simulink model "tb_drive_sys"  (R2026b)
settings: Solver=ode3  StopTime=1  FixedStep=1e-3  EnableMultiTasking=on
model workspace (MAT data in the model file):
  tb_J = 1.2798
  tb_Rsrc = 0.02
  tb_T_amb = 318.15
  tb_Trr = 6.97491
  tb_cmd.enable = timeseries
  tb_cmd.enable.Name = 'unnamed'
  tb_cmd.enable.DataInfo = tsdata.datametadata
  tb_cmd.enable.DataInfo.Interpolation = tsdata.interpolation
  tb_cmd.enable.DataInfo.Interpolation.Fhandle : function handle (value not decoded)
  tb_cmd.enable.DataInfo.Interpolation.Name = 'linear'
  tb_cmd.enable.TimeInfo = tsdata.timemetadata
  tb_cmd.enable.TimeInfo.Length = 1
  tb_cmd.enable.TimeInfo.DuplicateTimes = 0
  tb_cmd.enable.TimeInfo.Time_ = 0
  tb_cmd.enable.TimeInfo.Initialized = 1
  tb_cmd.enable.QualityInfo = tsdata.qualmetadata
  tb_cmd.enable.Data_ = 0
  tb_cmd.mode = timeseries
  tb_cmd.mode.Name = 'unnamed'
  tb_cmd.mode.DataInfo = tsdata.datametadata
  tb_cmd.mode.DataInfo.Interpolation = tsdata.interpolation
  tb_cmd.mode.DataInfo.Interpolation.Fhandle : function handle (value not decoded)
  tb_cmd.mode.DataInfo.Interpolation.Name = 'linear'
  tb_cmd.mode.TimeInfo = tsdata.timemetadata
  tb_cmd.mode.TimeInfo.Length = 1
  tb_cmd.mode.TimeInfo.DuplicateTimes = 0
  tb_cmd.mode.TimeInfo.Time_ = 0
  tb_cmd.mode.TimeInfo.Initialized = 1
  tb_cmd.mode.QualityInfo = tsdata.qualmetadata
  tb_cmd.mode.Data_ = 1
  tb_cmd.w_ref = timeseries
  tb_cmd.w_ref.Name = 'unnamed'
  tb_cmd.w_ref.DataInfo = tsdata.datametadata
  tb_cmd.w_ref.DataInfo.Interpolation = tsdata.interpolation
  tb_cmd.w_ref.DataInfo.Interpolation.Fhandle : function handle (value not decoded)
  tb_cmd.w_ref.DataInfo.Interpolation.Name = 'linear'
  tb_cmd.w_ref.TimeInfo = tsdata.timemetadata
  tb_cmd.w_ref.TimeInfo.Length = 1
  tb_cmd.w_ref.TimeInfo.DuplicateTimes = 0
  tb_cmd.w_ref.TimeInfo.Time_ = 0
  tb_cmd.w_ref.TimeInfo.Initialized = 1
  tb_cmd.w_ref.QualityInfo = tsdata.qualmetadata
  tb_cmd.w_ref.Data_ = 0
  tb_cmd.tau_ff = timeseries
  tb_cmd.tau_ff.Name = 'unnamed'
  tb_cmd.tau_ff.DataInfo = tsdata.datametadata
  tb_cmd.tau_ff.DataInfo.Interpolation = tsdata.interpolation
  tb_cmd.tau_ff.DataInfo.Interpolation.Fhandle : function handle (value not decoded)
  tb_cmd.tau_ff.DataInfo.Interpolation.Name = 'linear'
  tb_cmd.tau_ff.TimeInfo = tsdata.timemetadata
  tb_cmd.tau_ff.TimeInfo.Length = 1
  tb_cmd.tau_ff.TimeInfo.DuplicateTimes = 0
  tb_cmd.tau_ff.TimeInfo.Time_ = 0
  tb_cmd.tau_ff.TimeInfo.Initialized = 1
  tb_cmd.tau_ff.QualityInfo = tsdata.qualmetadata
  tb_cmd.tau_ff.Data_ = 0
  tb_cmd.tau_lim_mot = timeseries
  tb_cmd.tau_lim_mot.Name = 'unnamed'
  tb_cmd.tau_lim_mot.DataInfo = tsdata.datametadata
  tb_cmd.tau_lim_mot.DataInfo.Interpolation = tsdata.interpolation
  tb_cmd.tau_lim_mot.DataInfo.Interpolation.Fhandle : function handle (value not decoded)
  tb_cmd.tau_lim_mot.DataInfo.Interpolation.Name = 'linear'
  tb_cmd.tau_lim_mot.TimeInfo = tsdata.timemetadata
  tb_cmd.tau_lim_mot.TimeInfo.Length = 1
  tb_cmd.tau_lim_mot.TimeInfo.DuplicateTimes = 0
  tb_cmd.tau_lim_mot.TimeInfo.Time_ = 0
  tb_cmd.tau_lim_mot.TimeInfo.Initialized = 1
  tb_cmd.tau_lim_mot.QualityInfo = tsdata.qualmetadata
  tb_cmd.tau_lim_mot.Data_ = 16
  tb_cmd.tau_lim_reg = timeseries
  tb_cmd.tau_lim_reg.Name = 'unnamed'
  tb_cmd.tau_lim_reg.DataInfo = tsdata.datametadata
  tb_cmd.tau_lim_reg.DataInfo.Interpolation = tsdata.interpolation
  tb_cmd.tau_lim_reg.DataInfo.Interpolation.Fhandle : function handle (value not decoded)
  tb_cmd.tau_lim_reg.DataInfo.Interpolation.Name = 'linear'
  tb_cmd.tau_lim_reg.TimeInfo = tsdata.timemetadata
  tb_cmd.tau_lim_reg.TimeInfo.Length = 1
  tb_cmd.tau_lim_reg.TimeInfo.DuplicateTimes = 0
  tb_cmd.tau_lim_reg.TimeInfo.Time_ = 0
  tb_cmd.tau_lim_reg.TimeInfo.Initialized = 1
  tb_cmd.tau_lim_reg.QualityInfo = tsdata.qualmetadata
  tb_cmd.tau_lim_reg.Data_ = 16
  tb_cmd.park_req = timeseries
  tb_cmd.park_req.Name = 'unnamed'
  tb_cmd.park_req.DataInfo = tsdata.datametadata
  tb_cmd.park_req.DataInfo.Interpolation = tsdata.interpolation
  tb_cmd.park_req.DataInfo.Interpolation.Fhandle : function handle (value not decoded)
  tb_cmd.park_req.DataInfo.Interpolation.Name = 'linear'
  tb_cmd.park_req.TimeInfo = tsdata.timemetadata
  tb_cmd.park_req.TimeInfo.Length = 1
  tb_cmd.park_req.TimeInfo.DuplicateTimes = 0
  tb_cmd.park_req.TimeInfo.Time_ = 0
  tb_cmd.park_req.TimeInfo.Initialized = 1
  tb_cmd.park_req.QualityInfo = tsdata.qualmetadata
  tb_cmd.park_req.Data_ = 0
  tb_cmd.fault_reset = timeseries
  tb_cmd.fault_reset.Name = 'unnamed'
  tb_cmd.fault_reset.DataInfo = tsdata.datametadata
  tb_cmd.fault_reset.DataInfo.Interpolation = tsdata.interpolation
  tb_cmd.fault_reset.DataInfo.Interpolation.Fhandle : function handle (value not decoded)
  tb_cmd.fault_reset.DataInfo.Interpolation.Name = 'linear'
  tb_cmd.fault_reset.TimeInfo = tsdata.timemetadata
  tb_cmd.fault_reset.TimeInfo.Length = 1
  tb_cmd.fault_reset.TimeInfo.DuplicateTimes = 0
  tb_cmd.fault_reset.TimeInfo.Time_ = 0
  tb_cmd.fault_reset.TimeInfo.Initialized = 1
  tb_cmd.fault_reset.QualityInfo = tsdata.qualmetadata
  tb_cmd.fault_reset.Data_ = 0
  tb_cmd.alive = timeseries
  tb_cmd.alive.Name = 'unnamed'
  tb_cmd.alive.DataInfo = tsdata.datametadata
  tb_cmd.alive.DataInfo.Interpolation = tsdata.interpolation
  tb_cmd.alive.DataInfo.Interpolation.Fhandle : function handle (value not decoded)
  tb_cmd.alive.DataInfo.Interpolation.Name = 'linear'
  tb_cmd.alive.TimeInfo = tsdata.timemetadata
  tb_cmd.alive.TimeInfo.Length = 1
  tb_cmd.alive.TimeInfo.DuplicateTimes = 0
  tb_cmd.alive.TimeInfo.Time_ = 0
  tb_cmd.alive.TimeInfo.Initialized = 1
  tb_cmd.alive.QualityInfo = tsdata.qualmetadata
  tb_cmd.alive.Data_ = 0
  tb_cmdL.enable = timeseries
  tb_cmdL.enable.Name = 'unnamed'
  tb_cmdL.enable.DataInfo = tsdata.datametadata
  tb_cmdL.enable.DataInfo.Interpolation = tsdata.interpolation
  tb_cmdL.enable.DataInfo.Interpolation.Fhandle : function handle (value not decoded)
  tb_cmdL.enable.DataInfo.Interpolation.Name = 'linear'
  tb_cmdL.enable.TimeInfo = tsdata.timemetadata
  tb_cmdL.enable.TimeInfo.Length = 1
  tb_cmdL.enable.TimeInfo.DuplicateTimes = 0
  tb_cmdL.enable.TimeInfo.Time_ = 0
  tb_cmdL.enable.TimeInfo.Initialized = 1
  tb_cmdL.enable.QualityInfo = tsdata.qualmetadata
  tb_cmdL.enable.Data_ = 0
  tb_cmdL.mode = timeseries
  tb_cmdL.mode.Name = 'unnamed'
  tb_cmdL.mode.DataInfo = tsdata.datametadata
  tb_cmdL.mode.DataInfo.Interpolation = tsdata.interpolation
  tb_cmdL.mode.DataInfo.Interpolation.Fhandle : function handle (value not decoded)
  tb_cmdL.mode.DataInfo.Interpolation.Name = 'linear'
  tb_cmdL.mode.TimeInfo = tsdata.timemetadata
  tb_cmdL.mode.TimeInfo.Length = 1
  tb_cmdL.mode.TimeInfo.DuplicateTimes = 0
  tb_cmdL.mode.TimeInfo.Time_ = 0
  tb_cmdL.mode.TimeInfo.Initialized = 1
  tb_cmdL.mode.QualityInfo = tsdata.qualmetadata
  tb_cmdL.mode.Data_ = 1
  tb_cmdL.w_ref = timeseries
  tb_cmdL.w_ref.Name = 'unnamed'
  tb_cmdL.w_ref.DataInfo = tsdata.datametadata
  tb_cmdL.w_ref.DataInfo.Interpolation = tsdata.interpolation
  tb_cmdL.w_ref.DataInfo.Interpolation.Fhandle : function handle (value not decoded)
  tb_cmdL.w_ref.DataInfo.Interpolation.Name = 'linear'
  tb_cmdL.w_ref.TimeInfo = tsdata.timemetadata
  tb_cmdL.w_ref.TimeInfo.Length = 1
  tb_cmdL.w_ref.TimeInfo.DuplicateTimes = 0
  tb_cmdL.w_ref.TimeInfo.Time_ = 0
  tb_cmdL.w_ref.TimeInfo.Initialized = 1
  tb_cmdL.w_ref.QualityInfo = tsdata.qualmetadata
  tb_cmdL.w_ref.Data_ = 0
  tb_cmdL.tau_ff = timeseries
  tb_cmdL.tau_ff.Name = 'unnamed'
  tb_cmdL.tau_ff.DataInfo = tsdata.datametadata
  tb_cmdL.tau_ff.DataInfo.Interpolation = tsdata.interpolation
  tb_cmdL.tau_ff.DataInfo.Interpolation.Fhandle : function handle (value not decoded)
  tb_cmdL.tau_ff.DataInfo.Interpolation.Name = 'linear'
  tb_cmdL.tau_ff.TimeInfo = tsdata.timemetadata
  tb_cmdL.tau_ff.TimeInfo.Length = 1
  tb_cmdL.tau_ff.TimeInfo.DuplicateTimes = 0
  tb_cmdL.tau_ff.TimeInfo.Time_ = 0
  tb_cmdL.tau_ff.TimeInfo.Initialized = 1
  tb_cmdL.tau_ff.QualityInfo = tsdata.qualmetadata
  tb_cmdL.tau_ff.Data_ = 0
  tb_cmdL.tau_lim_mot = timeseries
  tb_cmdL.tau_lim_mot.Name = 'unnamed'
  tb_cmdL.tau_lim_mot.DataInfo = tsdata.datametadata
  tb_cmdL.tau_lim_mot.DataInfo.Interpolation = tsdata.interpolation
  tb_cmdL.tau_lim_mot.DataInfo.Interpolation.Fhandle : function handle (value not decoded)
  tb_cmdL.tau_lim_mot.DataInfo.Interpolation.Name = 'linear'
  tb_cmdL.tau_lim_mot.TimeInfo = tsdata.timemetadata
  tb_cmdL.tau_lim_mot.TimeInfo.Length = 1
  tb_cmdL.tau_lim_mot.TimeInfo.DuplicateTimes = 0
  tb_cmdL.tau_lim_mot.TimeInfo.Time_ = 0
  tb_cmdL.tau_lim_mot.TimeInfo.Initialized = 1
  tb_cmdL.tau_lim_mot.QualityInfo = tsdata.qualmetadata
  tb_cmdL.tau_lim_mot.Data_ = 16
  tb_cmdL.tau_lim_reg = timeseries
  tb_cmdL.tau_lim_reg.Name = 'unnamed'
  tb_cmdL.tau_lim_reg.DataInfo = tsdata.datametadata
  tb_cmdL.tau_lim_reg.DataInfo.Interpolation = tsdata.interpolation
  tb_cmdL.tau_lim_reg.DataInfo.Interpolation.Fhandle : function handle (value not decoded)
  tb_cmdL.tau_lim_reg.DataInfo.Interpolation.Name = 'linear'
  tb_cmdL.tau_lim_reg.TimeInfo = tsdata.timemetadata
  tb_cmdL.tau_lim_reg.TimeInfo.Length = 1
  tb_cmdL.tau_lim_reg.TimeInfo.DuplicateTimes = 0
  tb_cmdL.tau_lim_reg.TimeInfo.Time_ = 0
  tb_cmdL.tau_lim_reg.TimeInfo.Initialized = 1
  tb_cmdL.tau_lim_reg.QualityInfo = tsdata.qualmetadata
  tb_cmdL.tau_lim_reg.Data_ = 16
  tb_cmdL.park_req = timeseries
  tb_cmdL.park_req.Name = 'unnamed'
  tb_cmdL.park_req.DataInfo = tsdata.datametadata
  tb_cmdL.park_req.DataInfo.Interpolation = tsdata.interpolation
  tb_cmdL.park_req.DataInfo.Interpolation.Fhandle : function handle (value not decoded)
  tb_cmdL.park_req.DataInfo.Interpolation.Name = 'linear'
  tb_cmdL.park_req.TimeInfo = tsdata.timemetadata
  tb_cmdL.park_req.TimeInfo.Length = 1
  tb_cmdL.park_req.TimeInfo.DuplicateTimes = 0
  tb_cmdL.park_req.TimeInfo.Time_ = 0
  tb_cmdL.park_req.TimeInfo.Initialized = 1
  tb_cmdL.park_req.QualityInfo = tsdata.qualmetadata
  tb_cmdL.park_req.Data_ = 0
  tb_cmdL.fault_reset = timeseries
  tb_cmdL.fault_reset.Name = 'unnamed'
  tb_cmdL.fault_reset.DataInfo = tsdata.datametadata
  tb_cmdL.fault_reset.DataInfo.Interpolation = tsdata.interpolation
  tb_cmdL.fault_reset.DataInfo.Interpolation.Fhandle : function handle (value not decoded)
  tb_cmdL.fault_reset.DataInfo.Interpolation.Name = 'linear'
  tb_cmdL.fault_reset.TimeInfo = tsdata.timemetadata
  tb_cmdL.fault_reset.TimeInfo.Length = 1
  tb_cmdL.fault_reset.TimeInfo.DuplicateTimes = 0
  tb_cmdL.fault_reset.TimeInfo.Time_ = 0
  tb_cmdL.fault_reset.TimeInfo.Initialized = 1
  tb_cmdL.fault_reset.QualityInfo = tsdata.qualmetadata
  tb_cmdL.fault_reset.Data_ = 0
  tb_cmdL.alive = timeseries
  tb_cmdL.alive.Name = 'unnamed'
  tb_cmdL.alive.DataInfo = tsdata.datametadata
  tb_cmdL.alive.DataInfo.Interpolation = tsdata.interpolation
  tb_cmdL.alive.DataInfo.Interpolation.Fhandle : function handle (value not decoded)
  tb_cmdL.alive.DataInfo.Interpolation.Name = 'linear'
  tb_cmdL.alive.TimeInfo = tsdata.timemetadata
  tb_cmdL.alive.TimeInfo.Length = 1
  tb_cmdL.alive.TimeInfo.DuplicateTimes = 0
  tb_cmdL.alive.TimeInfo.Time_ = 0
  tb_cmdL.alive.TimeInfo.Initialized = 1
  tb_cmdL.alive.QualityInfo = tsdata.qualmetadata
  tb_cmdL.alive.Data_ = 0
  tb_cmdR.enable = timeseries
  tb_cmdR.enable.Name = 'unnamed'
  tb_cmdR.enable.DataInfo = tsdata.datametadata
  tb_cmdR.enable.DataInfo.Interpolation = tsdata.interpolation
  tb_cmdR.enable.DataInfo.Interpolation.Fhandle : function handle (value not decoded)
  tb_cmdR.enable.DataInfo.Interpolation.Name = 'linear'
  tb_cmdR.enable.TimeInfo = tsdata.timemetadata
  tb_cmdR.enable.TimeInfo.Length = 1
  tb_cmdR.enable.TimeInfo.DuplicateTimes = 0
  tb_cmdR.enable.TimeInfo.Time_ = 0
  tb_cmdR.enable.TimeInfo.Initialized = 1
  tb_cmdR.enable.QualityInfo = tsdata.qualmetadata
  tb_cmdR.enable.Data_ = 0
  tb_cmdR.mode = timeseries
  tb_cmdR.mode.Name = 'unnamed'
  tb_cmdR.mode.DataInfo = tsdata.datametadata
  tb_cmdR.mode.DataInfo.Interpolation = tsdata.interpolation
  tb_cmdR.mode.DataInfo.Interpolation.Fhandle : function handle (value not decoded)
  tb_cmdR.mode.DataInfo.Interpolation.Name = 'linear'
  tb_cmdR.mode.TimeInfo = tsdata.timemetadata
  tb_cmdR.mode.TimeInfo.Length = 1
  tb_cmdR.mode.TimeInfo.DuplicateTimes = 0
  tb_cmdR.mode.TimeInfo.Time_ = 0
  tb_cmdR.mode.TimeInfo.Initialized = 1
  tb_cmdR.mode.QualityInfo = tsdata.qualmetadata
  tb_cmdR.mode.Data_ = 1
  tb_cmdR.w_ref = timeseries
  tb_cmdR.w_ref.Name = 'unnamed'
  tb_cmdR.w_ref.DataInfo = tsdata.datametadata
  tb_cmdR.w_ref.DataInfo.Interpolation = tsdata.interpolation
  tb_cmdR.w_ref.DataInfo.Interpolation.Fhandle : function handle (value not decoded)
  tb_cmdR.w_ref.DataInfo.Interpolation.Name = 'linear'
  tb_cmdR.w_ref.TimeInfo = tsdata.timemetadata
  tb_cmdR.w_ref.TimeInfo.Length = 1
  tb_cmdR.w_ref.TimeInfo.DuplicateTimes = 0
  tb_cmdR.w_ref.TimeInfo.Time_ = 0
  tb_cmdR.w_ref.TimeInfo.Initialized = 1
  tb_cmdR.w_ref.QualityInfo = tsdata.qualmetadata
  tb_cmdR.w_ref.Data_ = 0
  tb_cmdR.tau_ff = timeseries
  tb_cmdR.tau_ff.Name = 'unnamed'
  tb_cmdR.tau_ff.DataInfo = tsdata.datametadata
  tb_cmdR.tau_ff.DataInfo.Interpolation = tsdata.interpolation
  tb_cmdR.tau_ff.DataInfo.Interpolation.Fhandle : function handle (value not decoded)
  tb_cmdR.tau_ff.DataInfo.Interpolation.Name = 'linear'
  tb_cmdR.tau_ff.TimeInfo = tsdata.timemetadata
  tb_cmdR.tau_ff.TimeInfo.Length = 1
  tb_cmdR.tau_ff.TimeInfo.DuplicateTimes = 0
  tb_cmdR.tau_ff.TimeInfo.Time_ = 0
  tb_cmdR.tau_ff.TimeInfo.Initialized = 1
  tb_cmdR.tau_ff.QualityInfo = tsdata.qualmetadata
  tb_cmdR.tau_ff.Data_ = 0
  tb_cmdR.tau_lim_mot = timeseries
  tb_cmdR.tau_lim_mot.Name = 'unnamed'
  tb_cmdR.tau_lim_mot.DataInfo = tsdata.datametadata
  tb_cmdR.tau_lim_mot.DataInfo.Interpolation = tsdata.interpolation
  tb_cmdR.tau_lim_mot.DataInfo.Interpolation.Fhandle : function handle (value not decoded)
  tb_cmdR.tau_lim_mot.DataInfo.Interpolation.Name = 'linear'
  tb_cmdR.tau_lim_mot.TimeInfo = tsdata.timemetadata
  tb_cmdR.tau_lim_mot.TimeInfo.Length = 1
  tb_cmdR.tau_lim_mot.TimeInfo.DuplicateTimes = 0
  tb_cmdR.tau_lim_mot.TimeInfo.Time_ = 0
  tb_cmdR.tau_lim_mot.TimeInfo.Initialized = 1
  tb_cmdR.tau_lim_mot.QualityInfo = tsdata.qualmetadata
  tb_cmdR.tau_lim_mot.Data_ = 16
  tb_cmdR.tau_lim_reg = timeseries
  tb_cmdR.tau_lim_reg.Name = 'unnamed'
  tb_cmdR.tau_lim_reg.DataInfo = tsdata.datametadata
  tb_cmdR.tau_lim_reg.DataInfo.Interpolation = tsdata.interpolation
  tb_cmdR.tau_lim_reg.DataInfo.Interpolation.Fhandle : function handle (value not decoded)
  tb_cmdR.tau_lim_reg.DataInfo.Interpolation.Name = 'linear'
  tb_cmdR.tau_lim_reg.TimeInfo = tsdata.timemetadata
  tb_cmdR.tau_lim_reg.TimeInfo.Length = 1
  tb_cmdR.tau_lim_reg.TimeInfo.DuplicateTimes = 0
  tb_cmdR.tau_lim_reg.TimeInfo.Time_ = 0
  tb_cmdR.tau_lim_reg.TimeInfo.Initialized = 1
  tb_cmdR.tau_lim_reg.QualityInfo = tsdata.qualmetadata
  tb_cmdR.tau_lim_reg.Data_ = 16
  tb_cmdR.park_req = timeseries
  tb_cmdR.park_req.Name = 'unnamed'
  tb_cmdR.park_req.DataInfo = tsdata.datametadata
  tb_cmdR.park_req.DataInfo.Interpolation = tsdata.interpolation
  tb_cmdR.park_req.DataInfo.Interpolation.Fhandle : function handle (value not decoded)
  tb_cmdR.park_req.DataInfo.Interpolation.Name = 'linear'
  tb_cmdR.park_req.TimeInfo = tsdata.timemetadata
  tb_cmdR.park_req.TimeInfo.Length = 1
  tb_cmdR.park_req.TimeInfo.DuplicateTimes = 0
  tb_cmdR.park_req.TimeInfo.Time_ = 0
  tb_cmdR.park_req.TimeInfo.Initialized = 1
  tb_cmdR.park_req.QualityInfo = tsdata.qualmetadata
  tb_cmdR.park_req.Data_ = 0
  tb_cmdR.fault_reset = timeseries
  tb_cmdR.fault_reset.Name = 'unnamed'
  tb_cmdR.fault_reset.DataInfo = tsdata.datametadata
  tb_cmdR.fault_reset.DataInfo.Interpolation = tsdata.interpolation
  tb_cmdR.fault_reset.DataInfo.Interpolation.Fhandle : function handle (value not decoded)
  tb_cmdR.fault_reset.DataInfo.Interpolation.Name = 'linear'
  tb_cmdR.fault_reset.TimeInfo = tsdata.timemetadata
  tb_cmdR.fault_reset.TimeInfo.Length = 1
  tb_cmdR.fault_reset.TimeInfo.DuplicateTimes = 0
  tb_cmdR.fault_reset.TimeInfo.Time_ = 0
  tb_cmdR.fault_reset.TimeInfo.Initialized = 1
  tb_cmdR.fault_reset.QualityInfo = tsdata.qualmetadata
  tb_cmdR.fault_reset.Data_ = 0
  tb_cmdR.alive = timeseries
  tb_cmdR.alive.Name = 'unnamed'
  tb_cmdR.alive.DataInfo = tsdata.datametadata
  tb_cmdR.alive.DataInfo.Interpolation = tsdata.interpolation
  tb_cmdR.alive.DataInfo.Interpolation.Fhandle : function handle (value not decoded)
  tb_cmdR.alive.DataInfo.Interpolation.Name = 'linear'
  tb_cmdR.alive.TimeInfo = tsdata.timemetadata
  tb_cmdR.alive.TimeInfo.Length = 1
  tb_cmdR.alive.TimeInfo.DuplicateTimes = 0
  tb_cmdR.alive.TimeInfo.Time_ = 0
  tb_cmdR.alive.TimeInfo.Initialized = 1
  tb_cmdR.alive.QualityInfo = tsdata.qualmetadata
  tb_cmdR.alive.Data_ = 0
  tb_contactor = timeseries
  tb_contactor.Name = 'unnamed'
  tb_contactor.DataInfo = tsdata.datametadata
  tb_contactor.DataInfo.Interpolation = tsdata.interpolation
  tb_contactor.DataInfo.Interpolation.Fhandle : function handle (value not decoded)
  tb_contactor.DataInfo.Interpolation.Name = 'linear'
  tb_contactor.TimeInfo = tsdata.timemetadata
  tb_contactor.TimeInfo.Length = 1
  tb_contactor.TimeInfo.DuplicateTimes = 0
  tb_contactor.TimeInfo.Time_ = 0
  tb_contactor.TimeInfo.Initialized = 1
  tb_contactor.QualityInfo = tsdata.qualmetadata
  tb_contactor.Data_ = 1
  tb_dec = 1
  tb_drop = timeseries
  tb_drop.Name = 'unnamed'
  tb_drop.DataInfo = tsdata.datametadata
  tb_drop.DataInfo.Interpolation = tsdata.interpolation
  tb_drop.DataInfo.Interpolation.Fhandle : function handle (value not decoded)
  tb_drop.DataInfo.Interpolation.Name = 'linear'
  tb_drop.TimeInfo = tsdata.timemetadata
  tb_drop.TimeInfo.Length = 1
  tb_drop.TimeInfo.DuplicateTimes = 0
  tb_drop.TimeInfo.Time_ = 0
  tb_drop.TimeInfo.Initialized = 1
  tb_drop.QualityInfo = tsdata.qualmetadata
  tb_drop.Data_ = 0
  tb_fi.L.can_drop = timeseries
  tb_fi.L.can_drop.Name = 'unnamed'
  tb_fi.L.can_drop.DataInfo = tsdata.datametadata
  tb_fi.L.can_drop.DataInfo.Interpolation = tsdata.interpolation
  tb_fi.L.can_drop.DataInfo.Interpolation.Fhandle : function handle (value not decoded)
  tb_fi.L.can_drop.DataInfo.Interpolation.Name = 'linear'
  tb_fi.L.can_drop.TimeInfo = tsdata.timemetadata
  tb_fi.L.can_drop.TimeInfo.Length = 1
  tb_fi.L.can_drop.TimeInfo.DuplicateTimes = 0
  tb_fi.L.can_drop.TimeInfo.Time_ = 0
  tb_fi.L.can_drop.TimeInfo.Initialized = 1
  tb_fi.L.can_drop.QualityInfo = tsdata.qualmetadata
  tb_fi.L.can_drop.Data_ = 0
  tb_fi.L.enc_fail = timeseries
  tb_fi.L.enc_fail.Name = 'unnamed'
  tb_fi.L.enc_fail.DataInfo = tsdata.datametadata
  tb_fi.L.enc_fail.DataInfo.Interpolation = tsdata.interpolation
  tb_fi.L.enc_fail.DataInfo.Interpolation.Fhandle : function handle (value not decoded)
  tb_fi.L.enc_fail.DataInfo.Interpolation.Name = 'linear'
  tb_fi.L.enc_fail.TimeInfo = tsdata.timemetadata
  tb_fi.L.enc_fail.TimeInfo.Length = 1
  tb_fi.L.enc_fail.TimeInfo.DuplicateTimes = 0
  tb_fi.L.enc_fail.TimeInfo.Time_ = 0
  tb_fi.L.enc_fail.TimeInfo.Initialized = 1
  tb_fi.L.enc_fail.QualityInfo = tsdata.qualmetadata
  tb_fi.L.enc_fail.Data_ = 0
  tb_fi.L.brake_stuck = timeseries
  tb_fi.L.brake_stuck.Name = 'unnamed'
  tb_fi.L.brake_stuck.DataInfo = tsdata.datametadata
  tb_fi.L.brake_stuck.DataInfo.Interpolation = tsdata.interpolation
  tb_fi.L.brake_stuck.DataInfo.Interpolation.Fhandle : function handle (value not decoded)
  tb_fi.L.brake_stuck.DataInfo.Interpolation.Name = 'linear'
  tb_fi.L.brake_stuck.TimeInfo = tsdata.timemetadata
  tb_fi.L.brake_stuck.TimeInfo.Length = 1
  tb_fi.L.brake_stuck.TimeInfo.DuplicateTimes = 0
  tb_fi.L.brake_stuck.TimeInfo.Time_ = 0
  tb_fi.L.brake_stuck.TimeInfo.Initialized = 1
  tb_fi.L.brake_stuck.QualityInfo = tsdata.qualmetadata
  tb_fi.L.brake_stuck.Data_ = 0
  tb_fi.L.tau_scale = timeseries
  tb_fi.L.tau_scale.Name = 'unnamed'
  tb_fi.L.tau_scale.DataInfo = tsdata.datametadata
  tb_fi.L.tau_scale.DataInfo.Interpolation = tsdata.interpolation
  tb_fi.L.tau_scale.DataInfo.Interpolation.Fhandle : function handle (value not decoded)
  tb_fi.L.tau_scale.DataInfo.Interpolation.Name = 'linear'
  tb_fi.L.tau_scale.TimeInfo = tsdata.timemetadata
  tb_fi.L.tau_scale.TimeInfo.Length = 1
  tb_fi.L.tau_scale.TimeInfo.DuplicateTimes = 0
  tb_fi.L.tau_scale.TimeInfo.Time_ = 0
  tb_fi.L.tau_scale.TimeInfo.Initialized = 1
  tb_fi.L.tau_scale.QualityInfo = tsdata.qualmetadata
  tb_fi.L.tau_scale.Data_ = 1
  tb_fi.L.T_offset = timeseries
  tb_fi.L.T_offset.Name = 'unnamed'
  tb_fi.L.T_offset.DataInfo = tsdata.datametadata
  tb_fi.L.T_offset.DataInfo.Interpolation = tsdata.interpolation
  tb_fi.L.T_offset.DataInfo.Interpolation.Fhandle : function handle (value not decoded)
  tb_fi.L.T_offset.DataInfo.Interpolation.Name = 'linear'
  tb_fi.L.T_offset.TimeInfo = tsdata.timemetadata
  tb_fi.L.T_offset.TimeInfo.Length = 1
  tb_fi.L.T_offset.TimeInfo.DuplicateTimes = 0
  tb_fi.L.T_offset.TimeInfo.Time_ = 0
  tb_fi.L.T_offset.TimeInfo.Initialized = 1
  tb_fi.L.T_offset.QualityInfo = tsdata.qualmetadata
  tb_fi.L.T_offset.Data_ = 0
  tb_fi.R.can_drop = timeseries
  tb_fi.R.can_drop.Name = 'unnamed'
  tb_fi.R.can_drop.DataInfo = tsdata.datametadata
  tb_fi.R.can_drop.DataInfo.Interpolation = tsdata.interpolation
  tb_fi.R.can_drop.DataInfo.Interpolation.Fhandle : function handle (value not decoded)
  tb_fi.R.can_drop.DataInfo.Interpolation.Name = 'linear'
  tb_fi.R.can_drop.TimeInfo = tsdata.timemetadata
  tb_fi.R.can_drop.TimeInfo.Length = 1
  tb_fi.R.can_drop.TimeInfo.DuplicateTimes = 0
  tb_fi.R.can_drop.TimeInfo.Time_ = 0
  tb_fi.R.can_drop.TimeInfo.Initialized = 1
  tb_fi.R.can_drop.QualityInfo = tsdata.qualmetadata
  tb_fi.R.can_drop.Data_ = 0
  tb_fi.R.enc_fail = timeseries
  tb_fi.R.enc_fail.Name = 'unnamed'
  tb_fi.R.enc_fail.DataInfo = tsdata.datametadata
  tb_fi.R.enc_fail.DataInfo.Interpolation = tsdata.interpolation
  tb_fi.R.enc_fail.DataInfo.Interpolation.Fhandle : function handle (value not decoded)
  tb_fi.R.enc_fail.DataInfo.Interpolation.Name = 'linear'
  tb_fi.R.enc_fail.TimeInfo = tsdata.timemetadata
  tb_fi.R.enc_fail.TimeInfo.Length = 1
  tb_fi.R.enc_fail.TimeInfo.DuplicateTimes = 0
  tb_fi.R.enc_fail.TimeInfo.Time_ = 0
  tb_fi.R.enc_fail.TimeInfo.Initialized = 1
  tb_fi.R.enc_fail.QualityInfo = tsdata.qualmetadata
  tb_fi.R.enc_fail.Data_ = 0
  tb_fi.R.brake_stuck = timeseries
  tb_fi.R.brake_stuck.Name = 'unnamed'
  tb_fi.R.brake_stuck.DataInfo = tsdata.datametadata
  tb_fi.R.brake_stuck.DataInfo.Interpolation = tsdata.interpolation
  tb_fi.R.brake_stuck.DataInfo.Interpolation.Fhandle : function handle (value not decoded)
  tb_fi.R.brake_stuck.DataInfo.Interpolation.Name = 'linear'
  tb_fi.R.brake_stuck.TimeInfo = tsdata.timemetadata
  tb_fi.R.brake_stuck.TimeInfo.Length = 1
  tb_fi.R.brake_stuck.TimeInfo.DuplicateTimes = 0
  tb_fi.R.brake_stuck.TimeInfo.Time_ = 0
  tb_fi.R.brake_stuck.TimeInfo.Initialized = 1
  tb_fi.R.brake_stuck.QualityInfo = tsdata.qualmetadata
  tb_fi.R.brake_stuck.Data_ = 0
  tb_fi.R.tau_scale = timeseries
  tb_fi.R.tau_scale.Name = 'unnamed'
  tb_fi.R.tau_scale.DataInfo = tsdata.datametadata
  tb_fi.R.tau_scale.DataInfo.Interpolation = tsdata.interpolation
  tb_fi.R.tau_scale.DataInfo.Interpolation.Fhandle : function handle (value not decoded)
  tb_fi.R.tau_scale.DataInfo.Interpolation.Name = 'linear'
  tb_fi.R.tau_scale.TimeInfo = tsdata.timemetadata
  tb_fi.R.tau_scale.TimeInfo.Length = 1
  tb_fi.R.tau_scale.TimeInfo.DuplicateTimes = 0
  tb_fi.R.tau_scale.TimeInfo.Time_ = 0
  tb_fi.R.tau_scale.TimeInfo.Initialized = 1
  tb_fi.R.tau_scale.QualityInfo = tsdata.qualmetadata
  tb_fi.R.tau_scale.Data_ = 1
  tb_fi.R.T_offset = timeseries
  tb_fi.R.T_offset.Name = 'unnamed'
  tb_fi.R.T_offset.DataInfo = tsdata.datametadata
  tb_fi.R.T_offset.DataInfo.Interpolation = tsdata.interpolation
  tb_fi.R.T_offset.DataInfo.Interpolation.Fhandle : function handle (value not decoded)
  tb_fi.R.T_offset.DataInfo.Interpolation.Name = 'linear'
  tb_fi.R.T_offset.TimeInfo = tsdata.timemetadata
  tb_fi.R.T_offset.TimeInfo.Length = 1
  tb_fi.R.T_offset.TimeInfo.DuplicateTimes = 0
  tb_fi.R.T_offset.TimeInfo.Time_ = 0
  tb_fi.R.T_offset.TimeInfo.Initialized = 1
  tb_fi.R.T_offset.QualityInfo = tsdata.qualmetadata
  tb_fi.R.T_offset.Data_ = 0
  tb_gradeL = timeseries
  tb_gradeL.Name = 'unnamed'
  tb_gradeL.DataInfo = tsdata.datametadata
  tb_gradeL.DataInfo.Interpolation = tsdata.interpolation
  tb_gradeL.DataInfo.Interpolation.Fhandle : function handle (value not decoded)
  tb_gradeL.DataInfo.Interpolation.Name = 'linear'
  tb_gradeL.TimeInfo = tsdata.timemetadata
  tb_gradeL.TimeInfo.Length = 1
  tb_gradeL.TimeInfo.DuplicateTimes = 0
  tb_gradeL.TimeInfo.Time_ = 0
  tb_gradeL.TimeInfo.Initialized = 1
  tb_gradeL.QualityInfo = tsdata.qualmetadata
  tb_gradeL.Data_ = 0
  tb_gradeR = timeseries
  tb_gradeR.Name = 'unnamed'
  tb_gradeR.DataInfo = tsdata.datametadata
  tb_gradeR.DataInfo.Interpolation = tsdata.interpolation
  tb_gradeR.DataInfo.Interpolation.Fhandle : function handle (value not decoded)
  tb_gradeR.DataInfo.Interpolation.Name = 'linear'
  tb_gradeR.TimeInfo = tsdata.timemetadata
  tb_gradeR.TimeInfo.Length = 1
  tb_gradeR.TimeInfo.DuplicateTimes = 0
  tb_gradeR.TimeInfo.Time_ = 0
  tb_gradeR.TimeInfo.Initialized = 1
  tb_gradeR.QualityInfo = tsdata.qualmetadata
  tb_gradeR.Data_ = 0
  tb_load = 1
  tb_sto = timeseries
  tb_sto.Name = 'unnamed'
  tb_sto.DataInfo = tsdata.datametadata
  tb_sto.DataInfo.Interpolation = tsdata.interpolation
  tb_sto.DataInfo.Interpolation.Fhandle : function handle (value not decoded)
  tb_sto.DataInfo.Interpolation.Name = 'linear'
  tb_sto.TimeInfo = tsdata.timemetadata
  tb_sto.TimeInfo.Length = 1
  tb_sto.TimeInfo.DuplicateTimes = 0
  tb_sto.TimeInfo.Time_ = 0
  tb_sto.TimeInfo.Initialized = 1
  tb_sto.QualityInfo = tsdata.qualmetadata
  tb_sto.Data_ = 1
  tb_vsrc = timeseries
  tb_vsrc.Name = 'unnamed'
  tb_vsrc.DataInfo = tsdata.datametadata
  tb_vsrc.DataInfo.Interpolation = tsdata.interpolation
  tb_vsrc.DataInfo.Interpolation.Fhandle : function handle (value not decoded)
  tb_vsrc.DataInfo.Interpolation.Name = 'linear'
  tb_vsrc.TimeInfo = tsdata.timemetadata
  tb_vsrc.TimeInfo.Length = 1
  tb_vsrc.TimeInfo.DuplicateTimes = 0
  tb_vsrc.TimeInfo.Time_ = 0
  tb_vsrc.TimeInfo.Initialized = 1
  tb_vsrc.QualityInfo = tsdata.qualmetadata
  tb_vsrc.Data_ = 46.8
values from neighbouring files (symbols this model uses):
  P = evalin('base', 'P')    [build_tb_drive.m]    (also in tb_drive_long.m; tb_drive_profile.m)
  Ts = tc.P.drive.Ts_esc    [t_drive.m]    (also in tb_drive_2mass_lti.m = P.drive.Ts_esc)
libraries: fl_lib x13, nesl_utility x5
settings Model: Creator=aomar  LastModifiedBy=aomar
settings ConfigSet: Description=Shaddad fixed-step 1 ms ode3, multitasking, explicit rate transitions (arch 7, D58).
settings DataIOCC: SignalLogging=off
settings OptimizationCC: SimCompilerOptimization=on
settings DebuggingCC: AlgebraicLoopMsg=error  ArtificialAlgebraicLoopMsg=error  SingleTaskRateTransMsg=error  StrictBusMsg=ErrorOnBusTreatedAsVector
settings SimscapeCC: SimscapeNominalValues="[{\"value\":\"1\",\"unit\":\"A\"},{\"value\":\"1\",\"unit\":\"bar\"},{\"value\":\"1\",\"unit\":\"cm^2\"},{\"value\":\"1\",\"unit\":\"cm^3/s\"},{\"value\":\"1\",\"unit\":\"kJ/kg\"},{\"value\":\"1\",\"unit\":\"kW\"},{\"value\":\"1\",\"unit\":\"l\"},{\"value\":\"1\",\"unit\":\"N\"},{\"value\":\"1\",\"unit\":\"N*m\"},{\"value\":\"1\",\"unit\":\"V\"},{\"value\":\"0.001\",\"unit\":\"Wb\"}]"  SimscapeNormalizeSystem=off  SimscapeUseEnergyAccounting=off

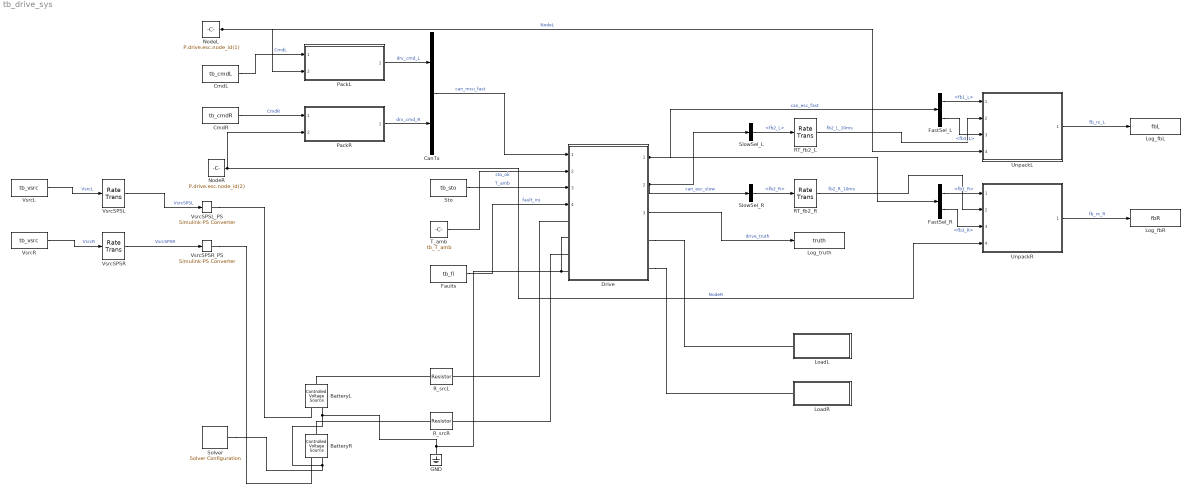
== system tb_drive_sys ==
  BatteryL : fl_lib/Electrical/Electrical Sources/Controlled Voltage Source
  BatteryR : fl_lib/Electrical/Electrical Sources/Controlled Voltage Source
  CanTx : BusCreator  Inputs=2  OutDataTypeStr=Bus: Bus_Can1_McuFast  NonVirtualBus=on
  CmdL : FromWorkspace  VariableName=tb_cmdL  OutDataTypeStr=Bus: Bus_DriveSideCmd  SampleTime=P.drive.Ts_can  Interpolate=off  OutputAfterFinalValue=Holding final value
  CmdR : FromWorkspace  VariableName=tb_cmdR  OutDataTypeStr=Bus: Bus_DriveSideCmd  SampleTime=P.drive.Ts_can  Interpolate=off  OutputAfterFinalValue=Holding final value
  Drive : Subsystem  ReferencedSubsystem=drive_system
  FastSel_L : BusSelector  OutputSignals=fb1_L,fb3_L
  FastSel_R : BusSelector  OutputSignals=fb1_R,fb3_R
  Faults : FromWorkspace  VariableName=tb_fi  OutDataTypeStr=Bus: Bus_DriveFaultInj  SampleTime=P.drive.Ts_esc  Interpolate=off  OutputAfterFinalValue=Holding final value
  GND : fl_lib/Electrical/Electrical Elements/Electrical Reference
  LoadL : Subsystem
  LoadR : Subsystem
  Log_fbL : ToWorkspace  VariableName=fbL  SaveFormat=Timeseries  SampleTime=-1
      settings: Decimation=tb_dec
  Log_fbR : ToWorkspace  VariableName=fbR  SaveFormat=Timeseries  SampleTime=-1
      settings: Decimation=tb_dec
  Log_truth : ToWorkspace  VariableName=truth  SaveFormat=Timeseries  SampleTime=-1
      settings: Decimation=tb_dec
  NodeL : Constant  Value=P.drive.esc.node_id(1)  OutDataTypeStr=uint8
  NodeR : Constant  Value=P.drive.esc.node_id(2)  OutDataTypeStr=uint8
  PackL : Subsystem  ReferencedSubsystem=drive_cmd_pack
  PackR : Subsystem  ReferencedSubsystem=drive_cmd_pack
  RT_fb2_L : RateTransition  OutPortSampleTime=P.drive.Ts_can
  RT_fb2_R : RateTransition  OutPortSampleTime=P.drive.Ts_can
  R_srcL : fl_lib/Electrical/Electrical Elements/Resistor  R=tb_Rsrc Ohm  i_specify=off  i_priority=None  i=0 A  i_nominal_specify=off  i_nominal_value=1  i_nominal_unit=A  v_specify=off  v_priority=None  v=0 V  v_nominal_specify=off  v_nominal_value=1  v_nominal_unit=V
  R_srcR : fl_lib/Electrical/Electrical Elements/Resistor  R=tb_Rsrc Ohm  i_specify=off  i_priority=None  i=0 A  i_nominal_specify=off  i_nominal_value=1  i_nominal_unit=A  v_specify=off  v_priority=None  v=0 V  v_nominal_specify=off  v_nominal_value=1  v_nominal_unit=V
  SlowSel_L : BusSelector  OutputSignals=fb2_L
  SlowSel_R : BusSelector  OutputSignals=fb2_R
  Solver : nesl_utility/Solver Configuration  PhysicalDomain=network_engine_domain  SubClassName=solver  LeftPortType=input  RightPortType=generic  Tones=[]  Harmonics=[]  SimulateNoise=off  Profile=off  UseLocalSampling=off  EnableSwitchedLinearOptims=on  FrequencyDomain=off  UseCCode=off  RelTol=0.001  AbsTol=0.001  MinStep=1e-09  ToWorkspace=off  RevertToSquareIcSolve=off  NumHomotopyIterations=100  PhasorMode=off  PhasorModeNumHarmonics=1  ConsistencySolver=NEWTON_XTOL_AFTER_FTOL  CanonicalOrdering=CANONICAL  OptimizeIntermediates=OPTIMIZED  MulticoreSolverChoice=BACKWARD_EULER  IndexReductionMethod=DerivativeReplacement  DoDC=off  ResidualTolerance=1e-09  ConsistencyTolSource=GLOBAL  ConsistencyAbsTol=0.001  ConsistencyRelTol=0.001  ConsistencyTolFactor=0.001  UseLocalSolver=on  LocalSolverChoice=NE_BACKWARD_EULER_ADVANCER  ResolveIndetEquations=on  FunctionEvalNumThread=1  LocalSolverSampleTime=P.sim.ssc.Ts  DoFixedCost=on  MaxNonlinIter=P.sim.ssc.MaxNonlinIter  MaxModeIter=P.sim.ssc.MaxModeIter  ComputeImpulses=off  ImpulseIterations=2  LinearAlgebra=auto  LinearAlgebraNumThread=0  EquationFormulation=NE_TIME_EF  DelaysMemoryBudget=1024  AutomaticFiltering=on  FilteringTimeConstant=0.001  PartitionStorageMethod=AS_NEEDED  PartitionMemoryBudget=1024  PartitionMethod=BALANCED  MultibodyUseLocalSolver=off  MultibodyLocalSolverChoice=ODE1  MultibodyLocalSolverSampleTime=0.001
  Sto : FromWorkspace  VariableName=tb_sto  OutDataTypeStr=boolean  SampleTime=P.drive.Ts_esc  Interpolate=off  OutputAfterFinalValue=Holding final value
  T_amb : Constant  Value=tb_T_amb  SampleTime=Ts.hk
  UnpackL : Subsystem  ReferencedSubsystem=drive_fb_unpack
  UnpackR : Subsystem  ReferencedSubsystem=drive_fb_unpack
  VsrcL : FromWorkspace  VariableName=tb_vsrc  SampleTime=P.drive.Ts_esc  Interpolate=off  OutputAfterFinalValue=Holding final value
  VsrcR : FromWorkspace  VariableName=tb_vsrc  SampleTime=P.drive.Ts_esc  Interpolate=off  OutputAfterFinalValue=Holding final value
  VsrcSPSL : RateTransition  OutPortSampleTimeOpt=Inherit
  VsrcSPSL_PS : nesl_utility/Simulink-PS Converter  PhysicalDomain=network_engine_domain  SubClassName=ps_input  LeftPortType=input  RightPortType=output  PseudoPeriodic=off  Frequencies=[]  NoiseDistribution=none  NoiseParameters=[]  Unit=V  AffineConversion=off  FilteringAndDerivatives=zero  SimscapeFilterOrder=1  InputFilterTimeConstant=0.001  UdotUserProvided=0
  VsrcSPSR : RateTransition  OutPortSampleTimeOpt=Inherit
  VsrcSPSR_PS : nesl_utility/Simulink-PS Converter  PhysicalDomain=network_engine_domain  SubClassName=ps_input  LeftPortType=input  RightPortType=output  PseudoPeriodic=off  Frequencies=[]  NoiseDistribution=none  NoiseParameters=[]  Unit=V  AffineConversion=off  FilteringAndDerivatives=zero  SimscapeFilterOrder=1  InputFilterTimeConstant=0.001  UdotUserProvided=0
  wires:
  VsrcL/1 -> VsrcSPSL/1  "VsrcL"
  VsrcR/1 -> VsrcSPSR/1  "VsrcR"
  VsrcSPSL/1 -> VsrcSPSL_PS/1  "VsrcSPSL"
  VsrcSPSR/1 -> VsrcSPSR_PS/1  "VsrcSPSR"
  NodeL/1 -> UnpackL/4, PackL/2  "NodeL"
  NodeR/1 -> UnpackR/4, PackR/2  "NodeR"
  CmdL/1 -> PackL/1  "CmdL"
  CmdR/1 -> PackR/1  "CmdR"
  PackL/1 -> CanTx/1  "drv_cmd_L"
  PackR/1 -> CanTx/2  "drv_cmd_R"
  CanTx/1 -> Drive/1  "can_mcu_fast"
  T_amb/1 -> Drive/3  "T_amb"
  Sto/1 -> Drive/2  "sto_ok"
  Faults/1 -> Drive/4  "fault_inj"
  Drive/1 -> FastSel_L/1, FastSel_R/1  "can_esc_fast"
  Drive/2 -> SlowSel_L/1, SlowSel_R/1  "can_esc_slow"
  Drive/3 -> Log_truth/1  "drive_truth"
  SlowSel_L/1 -> RT_fb2_L/1  "<fb2_L>"
  SlowSel_R/1 -> RT_fb2_R/1  "<fb2_R>"
  RT_fb2_L/1 -> UnpackL/2  "fb2_L_10ms"
  RT_fb2_R/1 -> UnpackR/2  "fb2_R_10ms"
  FastSel_L/1 -> UnpackL/1  "<fb1_L>"
  FastSel_L/2 -> UnpackL/3  "<fb3_L>"
  FastSel_R/1 -> UnpackR/1  "<fb1_R>"
  FastSel_R/2 -> UnpackR/3  "<fb3_R>"
  UnpackL/1 -> Log_fbL/1  "fb_rx_L"
  UnpackR/1 -> Log_fbR/1  "fb_rx_R"
  connections:
  BatteryL/LConn1 -- R_srcL/LConn1
  VsrcSPSL_PS/RConn1 -- BatteryL/RConn1
  BatteryR/RConn2 -- Solver/RConn1 -- BatteryL/RConn2 -- GND/LConn1 -- Drive/LConn4 -- Drive/LConn2
  BatteryR/LConn1 -- R_srcR/LConn1
  VsrcSPSR_PS/RConn1 -- BatteryR/RConn1
  Drive/LConn1 -- R_srcL/RConn1
  Drive/LConn3 -- R_srcR/RConn1
  Drive/RConn1 -- LoadL/LConn1
  Drive/RConn2 -- LoadR/LConn1

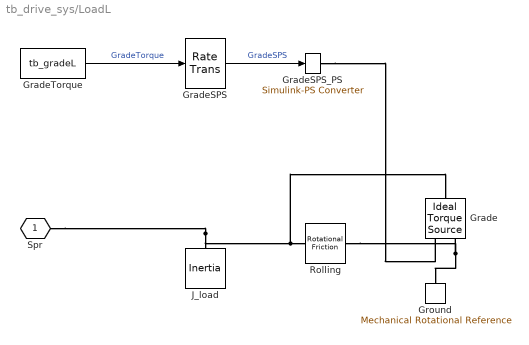
== system tb_drive_sys/LoadL ==
  Grade : fl_lib/Mechanical/Mechanical Sources/Ideal Torque Source
  GradeSPS : RateTransition  OutPortSampleTimeOpt=Inherit
  GradeSPS_PS : nesl_utility/Simulink-PS Converter  PhysicalDomain=network_engine_domain  SubClassName=ps_input  LeftPortType=input  RightPortType=output  PseudoPeriodic=off  Frequencies=[]  NoiseDistribution=none  NoiseParameters=[]  Unit=N*m  AffineConversion=off  FilteringAndDerivatives=zero  SimscapeFilterOrder=1  InputFilterTimeConstant=0.001  UdotUserProvided=0
  GradeTorque : FromWorkspace  VariableName=tb_gradeL  SampleTime=P.drive.Ts_esc  Interpolate=off  OutputAfterFinalValue=Holding final value
  Ground : fl_lib/Mechanical/Rotational Elements/Mechanical Rotational Reference
  J_load : fl_lib/Mechanical/Rotational Elements/Inertia  inertia=tb_J kg*m^2  num_ports=foundation.enum.numPorts2.one  w_specify=off  w_priority=High  w=0 rad/s  w_nominal_specify=off  w_nominal_value=1  w_nominal_unit=rad/s  t_specify=off  t_priority=None  t=0 N*m  t_nominal_specify=off  t_nominal_value=1  t_nominal_unit=N*m
  Rolling : fl_lib/Mechanical/Rotational Elements/Rotational Friction  brkwy_trq=1.0001*tb_Trr N*m  brkwy_vel=P.drive.bench.w_brk_rr rad/s  Col_trq=tb_Trr N*m  visc_coef=0 N*m*s/rad  w_specify=off  w_priority=None  w=0 rad/s  w_nominal_specify=off  w_nominal_value=1  w_nominal_unit=rad/s  t_specify=off  t_priority=None  t=0 N*m  t_nominal_specify=off  t_nominal_value=1  t_nominal_unit=N*m
  Spr : PMIOPort  Side=Left  ConnectionType=Connection: foundation.mechanical.rotational.rotational
  wires:
  GradeTorque/1 -> GradeSPS/1  "GradeTorque"
  GradeSPS/1 -> GradeSPS_PS/1  "GradeSPS"
  connections:
  J_load/LConn1 -- Spr/RConn1 -- Rolling/LConn1 -- Grade/LConn1
  GradeSPS_PS/RConn1 -- Grade/RConn1
  Grade/RConn2 -- Rolling/RConn1 -- Ground/LConn1

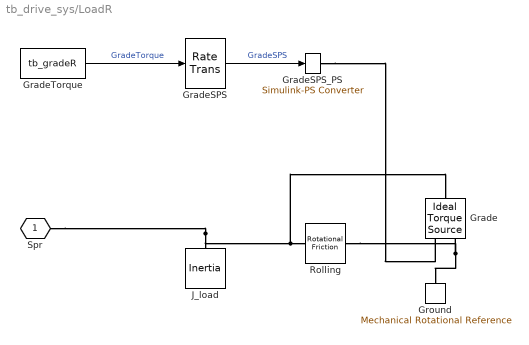
== system tb_drive_sys/LoadR ==
  Grade : fl_lib/Mechanical/Mechanical Sources/Ideal Torque Source
  GradeSPS : RateTransition  OutPortSampleTimeOpt=Inherit
  GradeSPS_PS : nesl_utility/Simulink-PS Converter  PhysicalDomain=network_engine_domain  SubClassName=ps_input  LeftPortType=input  RightPortType=output  PseudoPeriodic=off  Frequencies=[]  NoiseDistribution=none  NoiseParameters=[]  Unit=N*m  AffineConversion=off  FilteringAndDerivatives=zero  SimscapeFilterOrder=1  InputFilterTimeConstant=0.001  UdotUserProvided=0
  GradeTorque : FromWorkspace  VariableName=tb_gradeR  SampleTime=P.drive.Ts_esc  Interpolate=off  OutputAfterFinalValue=Holding final value
  Ground : fl_lib/Mechanical/Rotational Elements/Mechanical Rotational Reference
  J_load : fl_lib/Mechanical/Rotational Elements/Inertia  inertia=tb_J kg*m^2  num_ports=foundation.enum.numPorts2.one  w_specify=off  w_priority=High  w=0 rad/s  w_nominal_specify=off  w_nominal_value=1  w_nominal_unit=rad/s  t_specify=off  t_priority=None  t=0 N*m  t_nominal_specify=off  t_nominal_value=1  t_nominal_unit=N*m
  Rolling : fl_lib/Mechanical/Rotational Elements/Rotational Friction  brkwy_trq=1.0001*tb_Trr N*m  brkwy_vel=P.drive.bench.w_brk_rr rad/s  Col_trq=tb_Trr N*m  visc_coef=0 N*m*s/rad  w_specify=off  w_priority=None  w=0 rad/s  w_nominal_specify=off  w_nominal_value=1  w_nominal_unit=rad/s  t_specify=off  t_priority=None  t=0 N*m  t_nominal_specify=off  t_nominal_value=1  t_nominal_unit=N*m
  Spr : PMIOPort  Side=Left  ConnectionType=Connection: foundation.mechanical.rotational.rotational
  wires:
  GradeTorque/1 -> GradeSPS/1  "GradeTorque"
  GradeSPS/1 -> GradeSPS_PS/1  "GradeSPS"
  connections:
  J_load/LConn1 -- Spr/RConn1 -- Rolling/LConn1 -- Grade/LConn1
  GradeSPS_PS/RConn1 -- Grade/RConn1
  Grade/RConn2 -- Rolling/RConn1 -- Ground/LConn1
